simulink model "Fault detection in LVDC microgrid"  (R2025a)
settings: Solver=FixedStepDiscrete  StartTime=0.0  StopTime=0.2  FixedStep=1e-6  RelTol=1e-3
undefined symbols (not defined in the file): Acid, DiscIntNeverNeededParam, dspblkCoreblockFVToolHelper, gcbh, Lead
libraries: spsSeriesRLCBranchLib x17, simulink x15, spsIdealSwitchLib x10, spsGroundLib x8, spsCurrentMeasurementLib x6, simulink_extras x6, spsVoltageMeasurementLib x5, spsMosfetLib x3, spsPWMGeneratorDCDCLib x2, spsBatteryLib x1, spsDiodeLib x1, slpidlib x1
settings Model: Creator=karth  LastModifiedBy=karth

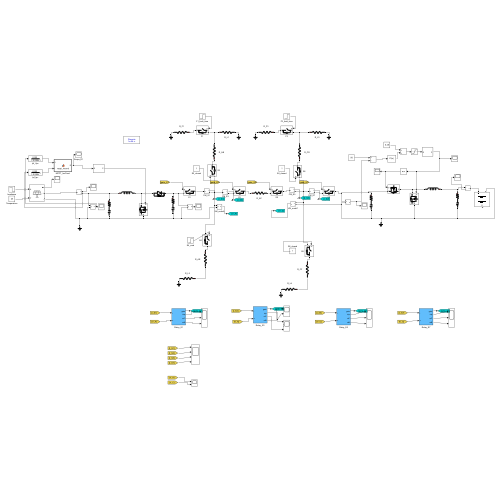
[thumbnail: Simulink's stored preview of the top-level diagram]
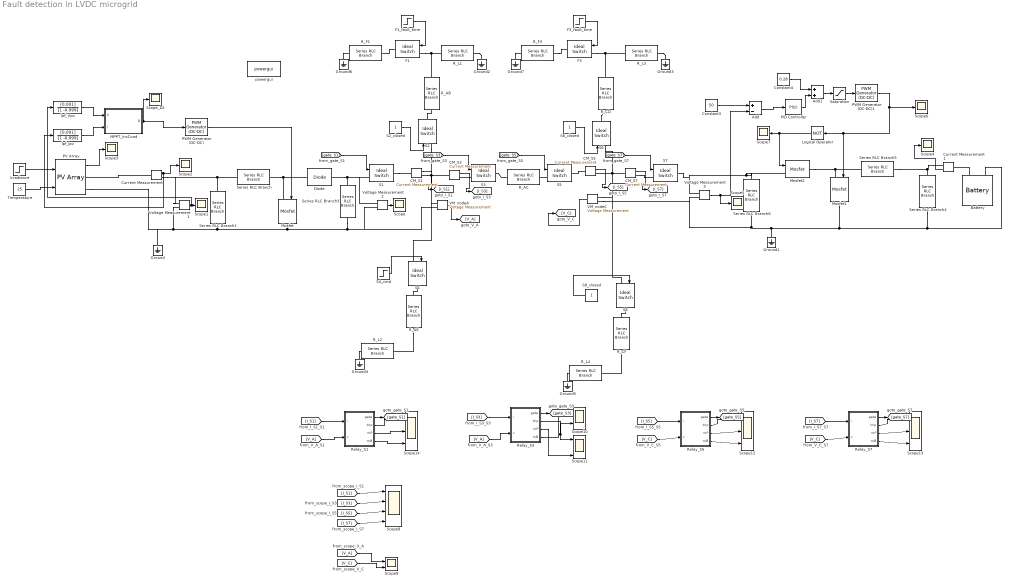
== system Fault detection in LVDC microgrid ==
  Add : Sum  Inputs=+-
  Add1 : Sum
  Battery : spsBatteryLib/Battery  BatType=Lead-Acid  NomV=36  NomQ=120  SOC=80  Batt_Tr=30  PresetModel=on  MaxQ=125  MinV=27  FullV=39.1974  Dis_rate=24  R=0.003  Normal_OP=37.2333  expZone="[36.6513          0.4]"
  CM_S{1,3,5,7} (4 alike) : spsCurrentMeasurementLib/Current Measurement  PhasorSimulation=off  OutputType=Complex  PSBequivalent=0
  Constant3 : Constant  Value=50
  Constant4 : Constant  Value=0.28
  Current Measurement : spsCurrentMeasurementLib/Current Measurement  PhasorSimulation=off  OutputType=Complex  PSBequivalent=0
  Current Measurement1 : spsCurrentMeasurementLib/Current Measurement  PhasorSimulation=off  OutputType=Complex  PSBequivalent=0
  Diode : spsDiodeLib/Diode  Ron=0.01  Lon=0  Vf=0.8  IC=0  UseSnubber=0  Rs=1e5  Cs=inf  Measurements=off
  F1 : spsIdealSwitchLib/Ideal Switch  Ron=1e-3  Lon=0  IC=0  Rs=1e6  Cs=inf  Measurements=off
  F1_fault_time : Step  Time=1000  SampleTime=1e-6
  F3 : spsIdealSwitchLib/Ideal Switch  Ron=1e-3  Lon=0  IC=0  Rs=1e6  Cs=inf  Measurements=off
  F3_fault_time : Step  Time=1000  SampleTime=1e-6
  Ground{,1..7} (8 alike) : spsGroundLib/Ground  LConnTagsString=a
  Irradiance : Step  Time=0.15  Before=700  After=50  SampleTime=1e-6
  Logical Operator : Logic  Operator=NOT  AllPortsSameDT=off  OutDataTypeStr=boolean
  MPPT_IncCond : MATLAB Function  TreatAsAtomicUnit=on
  Mosfet : spsMosfetLib/Mosfet  Ron=0.01  Lon=0  Rd=0.01  Vfd=0  IC=0  Rs=1e5  Cs=inf  Measurements=off
  Mosfet1 : spsMosfetLib/Mosfet  Ron=0.01  Lon=0  Rd=0.01  Vfd=0  IC=0  Rs=1e5  Cs=inf  Measurements=off
  Mosfet2 : spsMosfetLib/Mosfet  Ron=0.01  Lon=0  Rd=0.01  Vfd=0  IC=0  Rs=1e5  Cs=inf  Measurements=off
  PID Controller : slpidlib/PID Controller  Controller=PI  Form=Parallel  TimeDomain=Discrete-time  UseExternalTs=off  SampleTime=1e-4  IntegratorMethod=Forward Euler  FilterMethod=Forward Euler  ControllerParametersSource=internal  P=0  I=0.1  UseKiTs=off  D=0  UseExternalDerivativeSource=off  N=100  UseFilter=on  TunerSelectOption=Transfer Function Based (PID Tuner App)  InitialConditionSource=internal  InitialConditionForIntegrator=0  InitialConditionForFilter=0  DifferentiatorICPrevScaledInput=0  ExternalReset=none  TrackingMode=off  Kt=1  LimitOutput=off  SatLimitsSource=internal  UpperSaturationLimit=inf  LowerSaturationLimit=-inf  LinearizeAsGain=on  AntiWindupMode=none  Kb=1  LimitIntegrator=off  UpperIntegratorSaturationLimit=inf  LowerIntegratorSaturationLimit=-inf  POutMin=[]  POutMax=[]  IOutMin=[]  IOutMax=[]  DOutMin=[]  DOutMax=[]  NOutMin=[]  NOutMax=[]  SumOutMin=[]  SumOutMax=[]  SaturationOutMin=[]  SaturationOutMax=[]  PParamMin=[]  PParamMax=[]  IParamMin=[]  IParamMax=[]  DParamMin=[]  DParamMax=[]  NParamMin=[]  NParamMax=[]  KbParamMin=[]  KbParamMax=[]  KtParamMin=[]  KtParamMax=[]  KbOutMin=[]  KbOutMax=[]  KtOutMin=[]  KtOutMax=[]  IntegratorOutMin=[]  IntegratorOutMax=[]  FilterOutMin=[]  FilterOutMax=[]  SumI1OutMin=[]  SumI1OutMax=[]  SumI2OutMin=[]  SumI2OutMax=[]  SumI3OutMin=[]  SumI3OutMax=[]  SumI4OutMin=[]  SumI4OutMax=[]  SumDOutMin=[]  SumDOutMax=[]  DifferentiatorOutMin=[]  DifferentiatorOutMax=[]  FilterDiffOutCoefMin=[]  FilterDiffOutCoefMax=[]  ReciprocalOutMin=[]  ReciprocalOutMax=[]  SumDenOutMin=[]  SumDenOutMax=[]  SumNumOutMin=[]  SumNumOutMax=[]  DivideOutMin=[]  DivideOutMax=[]  UdiffTsProdOutMin=[]  UdiffTsProdOutMax=[]  NTsProdOutMin=[]  NTsProdOutMax=[]  UintegralTsProdOutMin=[]  UintegralTsProdOutMax=[]  UngainTsProdOutMin=[]  UngainTsProdOutMax=[]  ClampingZeroOutDataTypeStr=Inherit: Inherit via back propagation  ClampingZeroOutMin=[]  ClampingZeroOutMax=[]  FilterDenConstantOutDataTypeStr=Inherit: Inherit via back propagation  FilterDenConstantOutMin=[]  FilterDenConstantOutMax=[]  PCopyOutDataTypeStr=Inherit: Inherit via back propagation  PCopyOutMin=[]  PCopyOutMax=[]  NCopyOutDataTypeStr=Inherit: Inherit via back propagation  NCopyOutMin=[]  NCopyOutMax=[]  IntegratorContinuousStateAttributes=''  IntegratorStateMustResolveToSignalObject=off  IntegratorRTWStateStorageClass=Auto  FilterContinuousStateAttributes=''  FilterStateMustResolveToSignalObject=off  FilterRTWStateStorageClass=Auto  ParallelPVariant=InternalParameters  IdealPVariant=Disabled  IVariant=InternalParameters  DVariant=Disabled  IntegratorVariant=Discrete  SatVariant=Disabled  AWVariant=Passthrough  PCopyVariant=Disabled  TRVariant=Disabled  FdbkBlocksVariant=Forward  IdealPFdbkVariant=Disabled  SatFdbkVariant=Disabled  DerivativeFilterVariant=Disabled  NVariant=Disabled  NCopyVariant=Disabled_SignalSpec  FilterICVariant=Disabled  IntegratorICVariant=InternalICs  ExternalResetVariant=Disabled  TRSumVariant=Passthrough  SumFdbkVariant=Disabled  SumVariant=Sum_PI  TsampFilterVariant=InternalTs  TsampNgainVariant=Passthrough  TsampIntegralVariant=Disabled_SignalSpec  ExternalSaturationOutDataTypeStr=Inherit: Same as second input  DerivativeSourceVariant=Disabled  PreIntVariant=InternalPreInt
  PV Array : spsPVArrayLib/PV Array  Npar=1  Nser=1  PlotType=array @ 1000 W/m2 & specified temperatures  S_vec="[ 1000  500  100 ]"  Temp_C_vec="[ 45 25  ]"  ModuleName=User-defined  PlotWhenSelected=off  Pm=300  Ncell=60  Voc=37  Isc=10.5  Vm=30  Im=10  beta_Voc_pc=-0.36099  alpha_Isc_pc=0.102  beta_Voc=-0.13357  alpha_Isc=0.01071  IL=10.6016  I0=3.9458e-10  nI=0.99988  Rsh=377.7002  Rs=0.24698  RobustModel=off  RobustCellTemperature=313.3991  BAL=on  Tc=1e-6  Tfilter=5e-5
  PWM Generator (DC-DC) : spsPWMGeneratorDCDCLib/PWM Generator (DC-DC)  Fsw=20e3  Ts=1e-6
  PWM Generator (DC-DC)1 : spsPWMGeneratorDCDCLib/PWM Generator (DC-DC)  Fsw=20e3  Ts=1e-6
  R_AB : spsSeriesRLCBranchLib/Series RLC Branch  LConnTagsString=__new0  RConnTagsString=__new0  BranchType=R  Resistance=0.5  Inductance=1e-3  SetiL0=off  InitialCurrent=0  Capacitance=1e-6  Setx0=off  InitialVoltage=0  Measurements=None
  R_AC : spsSeriesRLCBranchLib/Series RLC Branch  LConnTagsString=__new0  RConnTagsString=__new0  BranchType=R  Resistance=0.5  Inductance=1e-3  SetiL0=off  InitialCurrent=0  Capacitance=1e-6  Setx0=off  InitialVoltage=0  Measurements=None
  R_AE : spsSeriesRLCBranchLib/Series RLC Branch  LConnTagsString=__new0  RConnTagsString=__new0  BranchType=R  Resistance=0.5  Inductance=1e-3  SetiL0=off  InitialCurrent=0  Capacitance=1e-6  Setx0=off  InitialVoltage=0  Measurements=None
  R_CD : spsSeriesRLCBranchLib/Series RLC Branch  LConnTagsString=__new0  RConnTagsString=__new0  BranchType=R  Resistance=0.5  Inductance=1e-3  SetiL0=off  InitialCurrent=0  Capacitance=1e-6  Setx0=off  InitialVoltage=0  Measurements=None
  R_CF : spsSeriesRLCBranchLib/Series RLC Branch  LConnTagsString=__new0  RConnTagsString=__new0  BranchType=R  Resistance=0.5  Inductance=1e-3  SetiL0=off  InitialCurrent=0  Capacitance=1e-6  Setx0=off  InitialVoltage=0  Measurements=None
  R_F1 : spsSeriesRLCBranchLib/Series RLC Branch  LConnTagsString=__new0  RConnTagsString=__new0  BranchType=R  Resistance=0.05  Inductance=1e-3  SetiL0=off  InitialCurrent=0  Capacitance=1e-6  Setx0=off  InitialVoltage=0  Measurements=None
  R_F3 : spsSeriesRLCBranchLib/Series RLC Branch  LConnTagsString=__new0  RConnTagsString=__new0  BranchType=R  Resistance=9.375  Inductance=1e-3  SetiL0=off  InitialCurrent=0  Capacitance=1e-6  Setx0=off  InitialVoltage=0  Measurements=None
  R_L{1..4} (4 alike) : spsSeriesRLCBranchLib/Series RLC Branch  LConnTagsString=__new0  RConnTagsString=__new0  BranchType=R  Resistance=50  Inductance=1e-3  SetiL0=off  InitialCurrent=0  Capacitance=1e-6  Setx0=off  InitialVoltage=0  Measurements=None
  Relay_S1 : Subsystem
  Relay_S3 : Subsystem
  Relay_S5 : Subsystem
  Relay_S7 : Subsystem
  S{1..8} (8 alike) : spsIdealSwitchLib/Ideal Switch  Ron=1e-3  Lon=0  IC=1  Rs=1e6  Cs=inf  Measurements=off
  S2_closed : Constant
  S4_cmd : Step  Time=1000  Before=1  SampleTime=1e-6
  S6_closed : Constant
  S8_closed : Constant
  Saturation : Saturate  UpperLimit=0.9  LowerLimit=0.05
  Scope{,1..7} (8 alike) : Scope
      Scope settings: ActiveDisplayYMinimum=46.814828818996375  ActiveDisplayYMaximum=55.3600246618051
      Scope1 settings: ActiveDisplayYMinimum=-103.67485509484459  ActiveDisplayYMaximum=435.433052683987
      Scope2 settings: ActiveDisplayYMinimum=4.4904226951960711  ActiveDisplayYMaximum=6.5640593859666954  DataLoggingVariableName=ScopeData2
      Scope3 settings: ActiveDisplayYMinimum=-103.67485509484459  ActiveDisplayYMaximum=435.433052683987  DataLoggingVariableName=ScopeData3
      Scope4 settings: ActiveDisplayYMinimum=-22.021538356838146  ActiveDisplayYMaximum=22.374841263668664  DataLoggingVariableName=ScopeData4
      Scope5 settings: ActiveDisplayYMinimum=34.063095110352663  ActiveDisplayYMaximum=89.684474056000283  DataLoggingVariableName=ScopeData5
      Scope6 settings: ActiveDisplayYMinimum=-3.7217195132358944  ActiveDisplayYMaximum=3.7132157718036125  DataLoggingVariableName=ScopeData6
      Scope7 settings: ActiveDisplayYMinimum=-0.31901661707500129  ActiveDisplayYMaximum=2.6002148529286919  DataLoggingVariableName=ScopeData7
  Scope10 : Scope  NumInputPorts=2
      settings: ActiveDisplayYMinimum=-5.0231938290397373  ActiveDisplayYMaximum=17.791992118445108  DataLoggingVariableName=ScopeData10
  Scope{11..14} (4 alike) : Scope  NumInputPorts=3
      Scope11 settings: ActiveDisplayYMinimum=-0.11029041288283192  ActiveDisplayYMaximum=1.0330501065949627  DataLoggingVariableName=ScopeData11
      Scope12 settings: ActiveDisplayYMinimum=-4.7472407047549252  ActiveDisplayYMaximum=8.8934108173964663  DataLoggingVariableName=ScopeData12
      Scope13 settings: ActiveDisplayYMinimum=-0.40971684709480044  ActiveDisplayYMaximum=0.45571135545856856  DataLoggingVariableName=ScopeData13
      Scope14 settings: ActiveDisplayYMinimum=0.0622817094865773  ActiveDisplayYMaximum=1.7514935531625646  DataLoggingVariableName=ScopeData13
  Scope8 : Scope  NumInputPorts=4
      settings: ActiveDisplayYMinimum=-17.983817604182249  ActiveDisplayYMaximum=137.21502473039885  DataLoggingVariableName=ScopeData8
  Scope9 : Scope  NumInputPorts=2
      settings: ActiveDisplayYMinimum=46.814828818996375  ActiveDisplayYMaximum=55.3600246618051  DataLoggingVariableName=ScopeData9
  Scope_D1 : Scope
      settings: ActiveDisplayYMinimum=0.39674693053993637  ActiveDisplayYMaximum=0.40749557339594983
  Series RLC Branch : spsSeriesRLCBranchLib/Series RLC Branch  LConnTagsString=__new0  RConnTagsString=__new0  BranchType=L  Resistance=1  Inductance=0.5e-3  SetiL0=off  InitialCurrent=0  Capacitance=1e-6  Setx0=off  InitialVoltage=0  Measurements=None
  Series RLC Branch1 : spsSeriesRLCBranchLib/Series RLC Branch  LConnTagsString=__new0  RConnTagsString=__new0  BranchType=RC  Resistance=0.1  Inductance=1e-3  SetiL0=off  InitialCurrent=0  Capacitance=470e-6  Setx0=on  InitialVoltage=30  Measurements=None
  Series RLC Branch3 : spsSeriesRLCBranchLib/Series RLC Branch  LConnTagsString=__new0  RConnTagsString=__new0  BranchType=RC  Resistance=0.2  Inductance=1e-3  SetiL0=off  InitialCurrent=0  Capacitance=470e-6  Setx0=on  InitialVoltage=50  Measurements=None
  Series RLC Branch4 : spsSeriesRLCBranchLib/Series RLC Branch  LConnTagsString=__new0  RConnTagsString=__new0  BranchType=RC  Resistance=0.05  Inductance=1e-3  SetiL0=off  InitialCurrent=0  Capacitance=470e-6  Setx0=on  InitialVoltage=36  Measurements=None
  Series RLC Branch5 : spsSeriesRLCBranchLib/Series RLC Branch  LConnTagsString=__new0  RConnTagsString=__new0  BranchType=L  Resistance=1  Inductance=1e-3  SetiL0=off  InitialCurrent=0  Capacitance=1e-6  Setx0=off  InitialVoltage=0  Measurements=None
  Series RLC Branch6 : spsSeriesRLCBranchLib/Series RLC Branch  LConnTagsString=__new0  RConnTagsString=__new0  BranchType=RC  Resistance=0.2  Inductance=1e-3  SetiL0=off  InitialCurrent=0  Capacitance=470e-6  Setx0=on  InitialVoltage=50  Measurements=None
  Temperature : Constant  Value=25
  VM_nodeA : spsVoltageMeasurementLib/Voltage Measurement  PhasorSimulation=off  OutputType=Complex  PSBequivalent=0
  VM_nodeC : spsVoltageMeasurementLib/Voltage Measurement  PhasorSimulation=off  OutputType=Complex  PSBequivalent=0
  Voltage Measurement1 : spsVoltageMeasurementLib/Voltage Measurement  PhasorSimulation=off  OutputType=Complex  PSBequivalent=0
  Voltage Measurement2 : spsVoltageMeasurementLib/Voltage Measurement  PhasorSimulation=off  OutputType=Complex  PSBequivalent=0
  Voltage Measurement3 : spsVoltageMeasurementLib/Voltage Measurement  PhasorSimulation=off  OutputType=Complex  PSBequivalent=0
  lpf_Ipv : DiscreteFilter  Numerator=[0.001]  Denominator=[1 -0.999]  SampleTime=1e-6
  lpf_Vpv : DiscreteFilter  Numerator=[0.001]  Denominator=[1 -0.999]  SampleTime=1e-6
  powergui : spspowerguiLib/powergui  Priority=1  SimulationMode=Discrete  SampleTime=1e-6  frequency=60  Iterations=50  frequencyindice=0  Pbase=100e6  ErrMax=1e-4  UnitsV=kV  UnitsW=MW  buscounter=0  FunctionMessages=off  echomessages=off  EnableUseOfTLC=off  CurrentSourceSwitches=off  DisableSnubberDevices=off  DisableRonSwitches=off  DisableVfSwitches=off  DisplayEquations=off  AutomaticDiscreteSolvers=off  SolverType=Tustin/Backward Euler (TBE)  Interpol=off  ExternalGateDelay=off  methode=off  Ts=100  x0status=blocks  SPID=on  SwTol=0  HookPort=off  NonlinearTolerance=1e-4  nMaxIteration=100  ContinueOnMaxIteration=off  RestoreLinks=warning  ResistiveCurrentMeasurement=off  Frange=[0:2:500]  Ylog=off  Xlog=on  ShowGrid=off  save=off  variable=ZData  structure=0  ZoomFFT=off  StartTime=0.0  cycles=1  DisplayStyle=1  fundamental=60  FreqAxis=off  MaxFrequency=1000  frequencyindicesteady=1  RmsSteady=1  display=off
  wires:
  PWM Generator (DC-DC)/1 -> Mosfet/1
  Irradiance/1 -> PV Array/1
  Temperature/1 -> PV Array/2
  Voltage Measurement2/1 -> Scope/1
  Voltage Measurement1/1 -> Scope1/1, lpf_Vpv/1
  Current Measurement/1 -> Scope2/1, lpf_Ipv/1
  PV Array/1 -> Scope3/1
  Current Measurement1/1 -> Scope4/1
  Constant3/1 -> Add/1
  Voltage Measurement3/1 -> Scope5/1, Add/2
  Add/1 -> PID Controller/1
  PID Controller/1 -> Add1/2
  PWM Generator (DC-DC)1/1 -> Mosfet1/1, Logical Operator/1, Scope6/1
  Logical Operator/1 -> Scope7/1, Mosfet2/1
  Add1/1 -> Saturation/1
  Constant4/1 -> Add1/1
  Saturation/1 -> PWM Generator (DC-DC)1/1
  S2_closed/1 -> S2/1
  S6_closed/1 -> S6/1
  S8_closed/1 -> S8/1
  F1_fault_time/1 -> F1/1
  F3_fault_time/1 -> F3/1
  Relay_S3/2(trip) -> Scope10/2, Scope11/1
  Relay_S3/3(mP) -> Scope11/3
  Relay_S3/4(mB) -> Scope10/1
  Relay_S5/2(trip) -> Scope12/1
  Relay_S5/3(mP) -> Scope12/2
  Relay_S5/4(mB) -> Scope12/3
  Relay_S7/2(trip) -> Scope13/1
  Relay_S7/3(mP) -> Scope13/2
  Relay_S7/4(mB) -> Scope13/3
  Relay_S1/2(trip) -> Scope14/1
  Relay_S1/3(mP) -> Scope14/2
  Relay_S1/4(mB) -> Scope14/3
  CM_S1/1 -> [I_S1]
  CM_S3/1 -> [I_S3]
  CM_S5/1 -> [I_S5]
  CM_S7/1 -> [I_S7]
  VM_nodeA/1 -> [V_A]
  VM_nodeC/1 -> [V_C]
  [I_S1] -> Relay_S1/1(i)
  [V_A] -> Relay_S1/2(v)
  Relay_S1/1(gate) -> [gate_S1]
  [I_S3] -> Relay_S3/1(i)
  [V_A] -> Relay_S3/2(v)
  Relay_S3/1(gate) -> [gate_S3]
  [I_S5] -> Relay_S5/1(i)
  [V_C] -> Relay_S5/2(v)
  Relay_S5/1(gate) -> [gate_S5]
  [I_S7] -> Relay_S7/1(i)
  [V_C] -> Relay_S7/2(v)
  Relay_S7/1(gate) -> [gate_S7]
  [gate_S1] -> S1/1
  [gate_S3] -> S3/1
  [gate_S5] -> S5/1
  [gate_S7] -> S7/1
  [I_S1] -> Scope8/1
  [I_S3] -> Scope8/2
  [I_S5] -> Scope8/3
  [I_S7] -> Scope8/4
  lpf_Vpv/1 -> MPPT_IncCond/1(V)
  lpf_Ipv/1 -> MPPT_IncCond/2(I)
  MPPT_IncCond/1(D) -> PWM Generator (DC-DC)/1, Scope_D1/1
  S4_cmd/1 -> S4/1
  [V_A] -> Scope9/1
  [V_C] -> Scope9/2
  connections:
  Series RLC Branch/LConn1 -- Voltage Measurement1/LConn1 -- Current Measurement/RConn1 -- Series RLC Branch1/LConn1
  Diode/LConn1 -- Mosfet/LConn1 -- Series RLC Branch/RConn1
  Mosfet2/LConn1 -- S7/RConn1 -- Voltage Measurement3/LConn1 -- Series RLC Branch6/LConn1
  Series RLC Branch1/RConn1 -- Ground/LConn1 -- PV Array/RConn2 -- Voltage Measurement1/LConn2 -- VM_nodeA/LConn2 -- Voltage Measurement2/LConn2 -- Series RLC Branch3/RConn1 -- Mosfet/RConn1
  Current Measurement/LConn1 -- PV Array/RConn1
  Series RLC Branch5/RConn1 -- Mosfet1/LConn1 -- Mosfet2/RConn1
  Battery/LConn2 -- Series RLC Branch4/RConn1 -- Mosfet1/RConn1 -- Ground1/LConn1 -- Voltage Measurement3/LConn2 -- VM_nodeC/LConn2 -- Series RLC Branch6/RConn1
  Battery/LConn1 -- Current Measurement1/LConn1
  Series RLC Branch5/LConn1 -- Series RLC Branch4/LConn1 -- Current Measurement1/RConn1
  Series RLC Branch3/LConn1 -- Voltage Measurement2/LConn1 -- S1/LConn1 -- Diode/RConn1
  R_AC/LConn1 -- S3/RConn1
  S5/LConn1 -- R_AC/RConn1
  S1/RConn1 -- CM_S1/LConn1
  S3/LConn1 -- CM_S3/RConn1
  CM_S1/RConn1 -- VM_nodeA/LConn1 -- S4/LConn1 -- CM_S3/LConn1 -- S2/LConn1
  CM_S5/LConn1 -- S5/RConn1
  CM_S7/LConn1 -- VM_nodeC/LConn1 -- S8/LConn1 -- CM_S5/RConn1 -- S6/LConn1
  CM_S7/RConn1 -- S7/LConn1
  S2/RConn1 -- R_AB/LConn1
  R_AB/RConn1 -- R_L1/LConn1 -- F1/LConn1
  R_L1/RConn1 -- Ground2/LConn1
  R_CD/RConn1 -- R_L3/LConn1 -- F3/LConn1
  S6/RConn1 -- R_CD/LConn1
  R_L3/RConn1 -- Ground3/LConn1
  R_AE/RConn1 -- R_L2/LConn1
  S4/RConn1 -- R_AE/LConn1
  Ground4/LConn1 -- R_L2/RConn1
  R_CF/RConn1 -- R_L4/LConn1
  Ground5/LConn1 -- R_L4/RConn1
  S8/RConn1 -- R_CF/LConn1
  R_F1/LConn1 -- F1/RConn1
  R_F1/RConn1 -- Ground6/LConn1
  R_F3/RConn1 -- Ground7/LConn1
  R_F3/LConn1 -- F3/RConn1

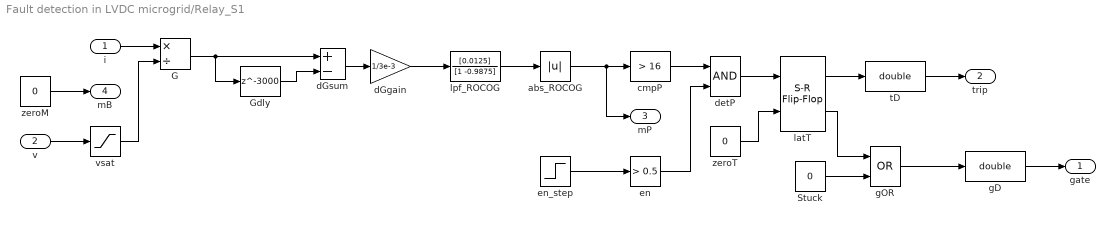
== system Fault detection in LVDC microgrid/Relay_S1 ==
  i : Inport
  v : Inport  Port=2
  G : Product  Inputs=*/
  Gdly : Delay  DelayLength=3000  InitialCondition=0  SampleTime=1e-6
  Stuck : Constant  Value=0  OutDataTypeStr=boolean
  abs_ROCOG : Abs
  cmpP : simulink/Logic and Bit Operations/Compare To Constant  relop=>  const=16  OutDataTypeStr=boolean
  dGgain : Gain  Gain=1/3e-3
  dGsum : Sum  Inputs=+-
  detP : Logic  AllPortsSameDT=off  OutDataTypeStr=boolean
  en : simulink/Logic and Bit Operations/Compare To Constant  relop=>  const=0.5  OutDataTypeStr=boolean
  en_step : Step  Time=0.08  SampleTime=1e-6
  gD : DataTypeConversion  OutDataTypeStr=double  SaturateOnIntegerOverflow=off  RndMeth=Floor
  gOR : Logic  Operator=OR  AllPortsSameDT=off  OutDataTypeStr=boolean
  latT : simulink_extras/Flip Flops/S-R Flip-Flop  initial_condition=0
  lpf_ROCOG : DiscreteFilter  LoadFcn=dspblkCoreblockFVToolHelper(gcbh,'load');  Numerator=[0.0125]  Denominator=[1 -0.9875]  SampleTime=1e-6
      settings: CopyFcn=dspblkCoreblockFVToolHelper(gcbh,'copy');  DeleteFcn=dspblkCoreblockFVToolHelper(gcbh,'close');  ModelCloseFcn=dspblkCoreblockFVToolHelper(gcbh,'close');  PreSaveFcn=dspblkCoreblockFVToolHelper(gcbh,'presave');  PostSaveFcn=dspblkCoreblockFVToolHelper(gcbh,'postsave');  CloseFcn=dspblkCoreblockFVToolHelper(gcbh,'close');
  tD : DataTypeConversion  OutDataTypeStr=double  SaturateOnIntegerOverflow=off  RndMeth=Floor
  vsat : Saturate  UpperLimit=1e6  LowerLimit=1e-3
  zeroM : Constant  Value=0
  zeroT : Constant  Value=0  OutDataTypeStr=boolean
  gate : Outport
  trip : Outport  Port=2
  mP : Outport  Port=3
  mB : Outport  Port=4
  wires:
  zeroM/1 -> mB/1
  G/1 -> dGsum/1, Gdly/1
  v/1 -> vsat/1
  dGgain/1 -> lpf_ROCOG/1
  i/1 -> G/1
  vsat/1 -> G/2
  gD/1 -> gate/1
  Gdly/1 -> dGsum/2
  detP/1 -> latT/1
  cmpP/1 -> detP/1
  dGsum/1 -> dGgain/1
  lpf_ROCOG/1 -> abs_ROCOG/1
  abs_ROCOG/1 -> cmpP/1, mP/1
  en_step/1 -> en/1
  en/1 -> detP/2
  zeroT/1 -> latT/2
  gOR/1 -> gD/1
  latT/1 -> tD/1
  latT/2 -> gOR/1
  Stuck/1 -> gOR/2
  tD/1 -> trip/1

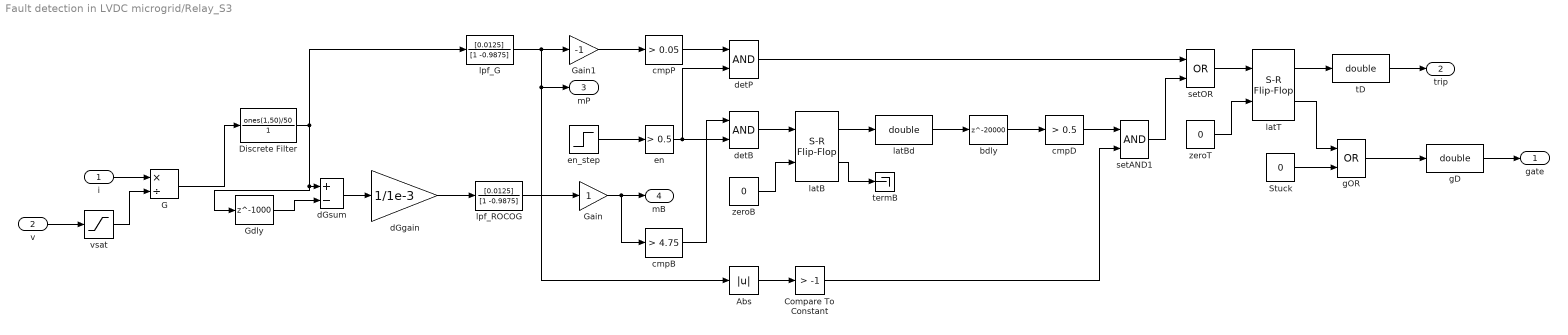
== system Fault detection in LVDC microgrid/Relay_S3 ==
  i : Inport
  v : Inport  Port=2
  Abs : Abs  SaturateOnIntegerOverflow=off
  Compare To Constant : simulink/Logic and Bit Operations/Compare To Constant  relop=>  const=-1  OutDataTypeStr=boolean
  Discrete Filter : DiscreteFilter  LoadFcn=dspblkCoreblockFVToolHelper(gcbh,'load');  Numerator=ones(1,50)/50  Denominator=1
      settings: CopyFcn=dspblkCoreblockFVToolHelper(gcbh,'copy');  DeleteFcn=dspblkCoreblockFVToolHelper(gcbh,'close');  ModelCloseFcn=dspblkCoreblockFVToolHelper(gcbh,'close');  PreSaveFcn=dspblkCoreblockFVToolHelper(gcbh,'presave');  PostSaveFcn=dspblkCoreblockFVToolHelper(gcbh,'postsave');  CloseFcn=dspblkCoreblockFVToolHelper(gcbh,'close');
  G : Product  Inputs=*/
  Gain : Gain
  Gain1 : Gain  Gain=-1
  Gdly : Delay  DelayLength=1000  InitialCondition=0  SampleTime=1e-6
  Stuck : Constant  Value=0  OutDataTypeStr=boolean
  bdly : Delay  DelayLength=20000  InitialCondition=0  SampleTime=1e-6
  cmpB : simulink/Logic and Bit Operations/Compare To Constant  relop=>  const=4.75  OutDataTypeStr=boolean
  cmpD : simulink/Logic and Bit Operations/Compare To Constant  relop=>  const=0.5  OutDataTypeStr=boolean
  cmpP : simulink/Logic and Bit Operations/Compare To Constant  relop=>  const=0.05  OutDataTypeStr=boolean
  dGgain : Gain  Gain=1/1e-3
  dGsum : Sum  Inputs=+-
  detB : Logic  AllPortsSameDT=off  OutDataTypeStr=boolean
  detP : Logic  AllPortsSameDT=off  OutDataTypeStr=boolean
  en : simulink/Logic and Bit Operations/Compare To Constant  relop=>  const=0.5  OutDataTypeStr=boolean
  en_step : Step  Time=0.08  SampleTime=1e-6
  gD : DataTypeConversion  OutDataTypeStr=double  SaturateOnIntegerOverflow=off  RndMeth=Floor
  gOR : Logic  Operator=OR  AllPortsSameDT=off  OutDataTypeStr=boolean
  latB : simulink_extras/Flip Flops/S-R Flip-Flop  initial_condition=0
  latBd : DataTypeConversion  OutDataTypeStr=double  SaturateOnIntegerOverflow=off  RndMeth=Floor
  latT : simulink_extras/Flip Flops/S-R Flip-Flop  initial_condition=0
  lpf_G : DiscreteFilter  Numerator=[0.0125]  Denominator=[1 -0.9875]  SampleTime=1e-6
  lpf_ROCOG : DiscreteFilter  Numerator=[0.0125]  Denominator=[1 -0.9875]  SampleTime=1e-6
  setAND1 : Logic  AllPortsSameDT=off  OutDataTypeStr=boolean
  setOR : Logic  Operator=OR  AllPortsSameDT=off  OutDataTypeStr=boolean
  tD : DataTypeConversion  OutDataTypeStr=double  SaturateOnIntegerOverflow=off  RndMeth=Floor
  termB : Terminator
  vsat : Saturate  UpperLimit=1e6  LowerLimit=1e-3
  zeroB : Constant  Value=0  OutDataTypeStr=boolean
  zeroT : Constant  Value=0  OutDataTypeStr=boolean
  gate : Outport
  trip : Outport  Port=2
  mP : Outport  Port=3
  mB : Outport  Port=4
  wires:
  dGgain/1 -> lpf_ROCOG/1
  cmpB/1 -> detB/1
  Gdly/1 -> dGsum/2
  Stuck/1 -> gOR/2
  i/1 -> G/1
  cmpP/1 -> detP/1
  v/1 -> vsat/1
  lpf_G/1 -> Abs/1, mP/1, Gain1/1
  setOR/1 -> latT/1
  vsat/1 -> G/2
  gD/1 -> gate/1
  latB/1 -> latBd/1
  detP/1 -> setOR/1
  dGsum/1 -> dGgain/1
  zeroT/1 -> latT/2
  lpf_ROCOG/1 -> Gain/1
  gOR/1 -> gD/1
  latBd/1 -> bdly/1
  detB/1 -> latB/1
  Gain1/1 -> cmpP/1
  en_step/1 -> en/1
  bdly/1 -> cmpD/1
  Gain/1 -> cmpB/1, mB/1
  en/1 -> detP/2, detB/2
  zeroB/1 -> latB/2
  Abs/1 -> Compare To Constant/1
  latB/2 -> termB/1
  Compare To Constant/1 -> setAND1/2
  cmpD/1 -> setAND1/1
  setAND1/1 -> setOR/2
  latT/1 -> tD/1
  latT/2 -> gOR/1
  tD/1 -> trip/1
  G/1 -> Discrete Filter/1
  Discrete Filter/1 -> dGsum/1, Gdly/1, lpf_G/1

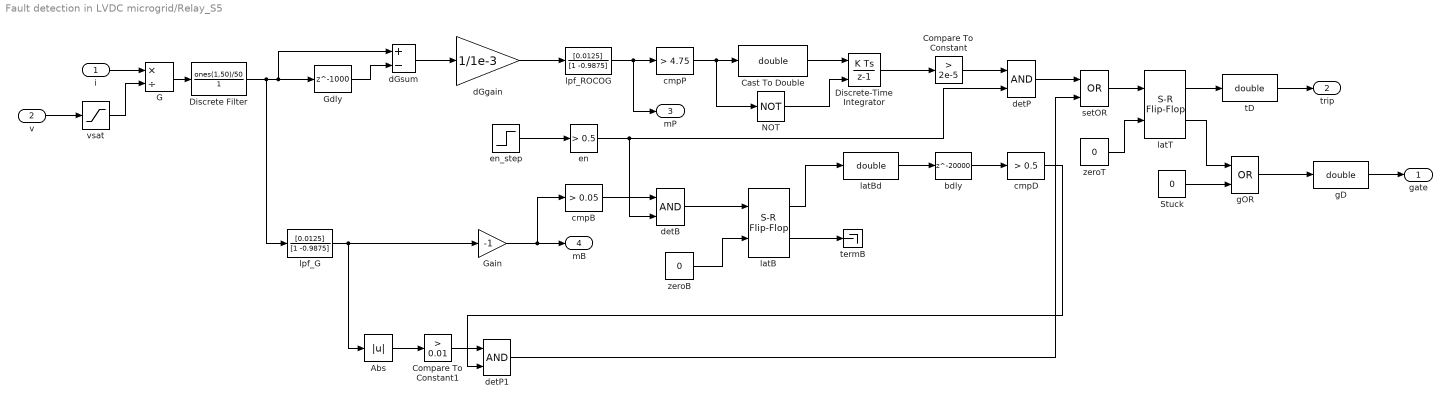
== system Fault detection in LVDC microgrid/Relay_S5 ==
  i : Inport
  v : Inport  Port=2
  Abs : Abs  SaturateOnIntegerOverflow=off
  Cast To Double : DataTypeConversion  OutDataTypeStr=double  SaturateOnIntegerOverflow=off  RndMeth=Floor
  Compare To Constant : simulink/Logic and Bit Operations/Compare To Constant  relop=>  const=2e-5  OutDataTypeStr=boolean
  Compare To Constant1 : simulink/Logic and Bit Operations/Compare To Constant  relop=>  const=0.01  OutDataTypeStr=boolean
  Discrete Filter : DiscreteFilter  LoadFcn=dspblkCoreblockFVToolHelper(gcbh,'load');  Numerator=ones(1,50)/50  Denominator=1
      settings: CopyFcn=dspblkCoreblockFVToolHelper(gcbh,'copy');  DeleteFcn=dspblkCoreblockFVToolHelper(gcbh,'close');  ModelCloseFcn=dspblkCoreblockFVToolHelper(gcbh,'close');  PreSaveFcn=dspblkCoreblockFVToolHelper(gcbh,'presave');  PostSaveFcn=dspblkCoreblockFVToolHelper(gcbh,'postsave');  CloseFcn=dspblkCoreblockFVToolHelper(gcbh,'close');
  Discrete-Time Integrator : DiscreteIntegrator  ExternalReset=level  SampleTime=1e-6  ICPrevOutput=DiscIntNeverNeededParam  ICPrevScaledInput=DiscIntNeverNeededParam
  G : Product  Inputs=*/
  Gain : Gain  Gain=-1
  Gdly : Delay  DelayLength=1000  InitialCondition=0  SampleTime=1e-6
  NOT : Logic  Operator=NOT  IconShape=distinctive  AllPortsSameDT=off  OutDataTypeStr=boolean
  Stuck : Constant  Value=0  OutDataTypeStr=boolean
  bdly : Delay  DelayLength=20000  InitialCondition=0  SampleTime=1e-6
  cmpB : simulink/Logic and Bit Operations/Compare To Constant  relop=>  const=0.05  OutDataTypeStr=boolean
  cmpD : simulink/Logic and Bit Operations/Compare To Constant  relop=>  const=0.5  OutDataTypeStr=boolean
  cmpP : simulink/Logic and Bit Operations/Compare To Constant  relop=>  const=4.75  OutDataTypeStr=boolean
  dGgain : Gain  Gain=1/1e-3
  dGsum : Sum  Inputs=+-
  detB : Logic  AllPortsSameDT=off  OutDataTypeStr=boolean
  detP : Logic  AllPortsSameDT=off  OutDataTypeStr=boolean
  detP1 : Logic  AllPortsSameDT=off  OutDataTypeStr=boolean
  en : simulink/Logic and Bit Operations/Compare To Constant  relop=>  const=0.5  OutDataTypeStr=boolean
  en_step : Step  Time=0.08  SampleTime=1e-6
  gD : DataTypeConversion  OutDataTypeStr=double  SaturateOnIntegerOverflow=off  RndMeth=Floor
  gOR : Logic  Operator=OR  AllPortsSameDT=off  OutDataTypeStr=boolean
  latB : simulink_extras/Flip Flops/S-R Flip-Flop  initial_condition=0
  latBd : DataTypeConversion  OutDataTypeStr=double  SaturateOnIntegerOverflow=off  RndMeth=Floor
  latT : simulink_extras/Flip Flops/S-R Flip-Flop  initial_condition=0
  lpf_G : DiscreteFilter  Numerator=[0.0125]  Denominator=[1 -0.9875]  SampleTime=1e-6
  lpf_ROCOG : DiscreteFilter  Numerator=[0.0125]  Denominator=[1 -0.9875]  SampleTime=1e-6
  setOR : Logic  Operator=OR  AllPortsSameDT=off  OutDataTypeStr=boolean
  tD : DataTypeConversion  OutDataTypeStr=double  SaturateOnIntegerOverflow=off  RndMeth=Floor
  termB : Terminator
  vsat : Saturate  UpperLimit=1e6  LowerLimit=1e-3
  zeroB : Constant  Value=0  OutDataTypeStr=boolean
  zeroT : Constant  Value=0  OutDataTypeStr=boolean
  gate : Outport
  trip : Outport  Port=2
  mP : Outport  Port=3
  mB : Outport  Port=4
  wires:
  Compare To Constant/1 -> detP/1
  i/1 -> G/1
  v/1 -> vsat/1
  setOR/1 -> latT/1
  vsat/1 -> G/2
  NOT/1 -> Discrete-Time Integrator/2
  dGgain/1 -> lpf_ROCOG/1
  bdly/1 -> cmpD/1
  Gdly/1 -> dGsum/2
  gD/1 -> gate/1
  detP/1 -> setOR/1
  latB/1 -> latBd/1
  dGsum/1 -> dGgain/1
  en_step/1 -> en/1
  Stuck/1 -> gOR/2
  Gain/1 -> cmpB/1, mB/1
  zeroT/1 -> latT/2
  lpf_ROCOG/1 -> mP/1, cmpP/1
  en/1 -> detP/2, detB/2
  cmpB/1 -> detB/1
  cmpP/1 -> NOT/1, Cast To Double/1
  gOR/1 -> gD/1
  latBd/1 -> bdly/1
  detB/1 -> latB/1
  zeroB/1 -> latB/2
  Cast To Double/1 -> Discrete-Time Integrator/1
  latB/2 -> termB/1
  Discrete-Time Integrator/1 -> Compare To Constant/1
  latT/1 -> tD/1
  latT/2 -> gOR/1
  tD/1 -> trip/1
  G/1 -> Discrete Filter/1
  Discrete Filter/1 -> lpf_G/1, dGsum/1, Gdly/1
  Abs/1 -> Compare To Constant1/1
  lpf_G/1 -> Abs/1, Gain/1
  Compare To Constant1/1 -> detP1/2
  cmpD/1 -> detP1/1
  detP1/1 -> setOR/2

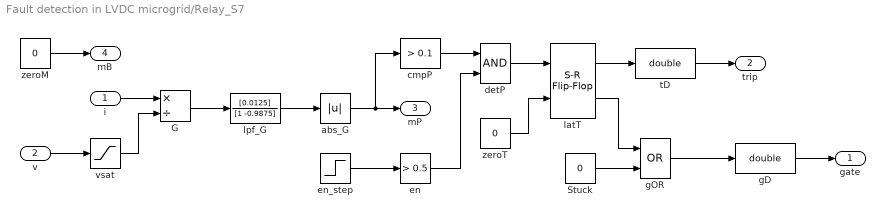
== system Fault detection in LVDC microgrid/Relay_S7 ==
  i : Inport
  v : Inport  Port=2
  G : Product  Inputs=*/
  Stuck : Constant  Value=0  OutDataTypeStr=boolean
  abs_G : Abs
  cmpP : simulink/Logic and Bit Operations/Compare To Constant  relop=>  const=0.1  OutDataTypeStr=boolean
  detP : Logic  AllPortsSameDT=off  OutDataTypeStr=boolean
  en : simulink/Logic and Bit Operations/Compare To Constant  relop=>  const=0.5  OutDataTypeStr=boolean
  en_step : Step  Time=0.08  SampleTime=1e-6
  gD : DataTypeConversion  OutDataTypeStr=double  SaturateOnIntegerOverflow=off  RndMeth=Floor
  gOR : Logic  Operator=OR  AllPortsSameDT=off  OutDataTypeStr=boolean
  latT : simulink_extras/Flip Flops/S-R Flip-Flop  initial_condition=0
  lpf_G : DiscreteFilter  Numerator=[0.0125]  Denominator=[1 -0.9875]  SampleTime=1e-6
  tD : DataTypeConversion  OutDataTypeStr=double  SaturateOnIntegerOverflow=off  RndMeth=Floor
  vsat : Saturate  UpperLimit=1e6  LowerLimit=1e-3
  zeroM : Constant  Value=0
  zeroT : Constant  Value=0  OutDataTypeStr=boolean
  gate : Outport
  trip : Outport  Port=2
  mP : Outport  Port=3
  mB : Outport  Port=4
  wires:
  vsat/1 -> G/2
  zeroM/1 -> mB/1
  G/1 -> lpf_G/1
  Stuck/1 -> gOR/2
  i/1 -> G/1
  v/1 -> vsat/1
  en_step/1 -> en/1
  latT/2 -> gOR/1
  abs_G/1 -> cmpP/1, mP/1
  gOR/1 -> gD/1
  cmpP/1 -> detP/1
  lpf_G/1 -> abs_G/1
  en/1 -> detP/2
  gD/1 -> gate/1
  latT/1 -> tD/1
  detP/1 -> latT/1
  zeroT/1 -> latT/2
  tD/1 -> trip/1

== matlab function Fault detection in LVDC microgrid/MPPT_IncCond ==
  settings: updateMethod=DISCRETE  sampleTime=0.01
  data: V input; D output; I input
function D = mppt_incond(V, I)
% Incremental-conductance MPPT. Boost: V_pv = V_bus*(1-D).
dD = 0.002; Dmin = 0.1; Dmax = 0.8; D0 = 0.4; tol = 0.01;
persistent Vp Ip Dk
if isempty(Vp), Vp = V; Ip = I; Dk = D0; end
dV = V - Vp;  dI = I - Ip;
if abs(dV) < 1e-3
    if dI > 1e-3,      Dk = Dk - dD;
    elseif dI < -1e-3, Dk = Dk + dD;
    end
else
    e = dI/dV + I/max(V, 1e-3);   % >0: left of MPP
    if e > tol,        Dk = Dk - dD;
    elseif e < -tol,   Dk = Dk + dD;
    end
end
Dk = min(max(Dk, Dmin), Dmax);
Vp = V; Ip = I; D = Dk;
